simulink library "lib_SecCtrl_Matrices1"  (R2026a)
settings: Solver=VariableStepAuto
undefined symbols (not defined in the file): A_f_sc, A_P_sc, A_Q_sc, A_v_sc, buses_lf, costs2, passM, sec_control_structure
libraries: simulink x3, sl_discontinuities x2
settings Model: Creator=atomas  LastModifiedBy=atomas

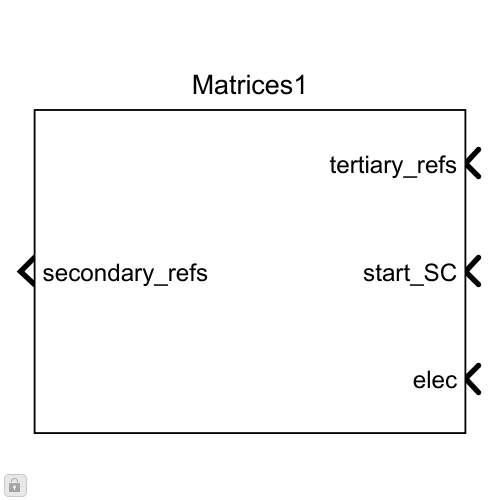
[thumbnail: Simulink's stored preview of the top-level diagram]
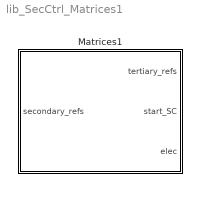
== system lib_SecCtrl_Matrices1 ==
  Matrices1 : Subsystem  VariantControl=Matrices1

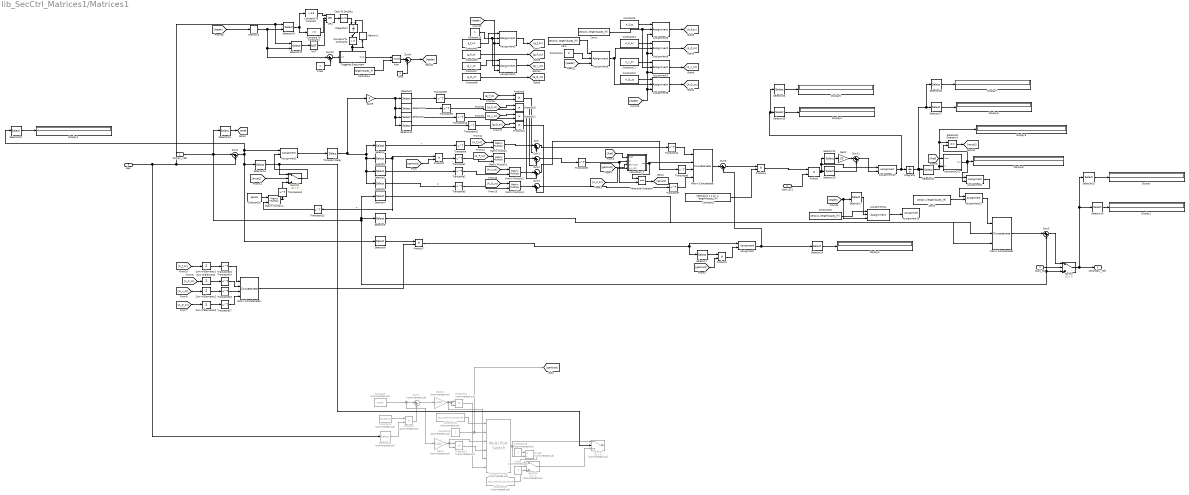
== system lib_SecCtrl_Matrices1/Matrices1 ==
  tertiary_refs : Inport
  start_SC : Inport  Port=2
  elec : Inport  Port=3
  Assignment{,1..2,13} (4 alike) : Assignment  NumberOfDimensions=2  DiagnosticForDimensions=Warning  IndexOptions=Index vector (dialog),Assign all  Indices=2,1  OutputSizes=1,1
  Assignment10 : Assignment  NumberOfDimensions=2  DiagnosticForDimensions=Warning  IndexOptions=Index vector (dialog),Assign all  Indices=1,1  OutputSizes=1,1
  Assignment{3..4,9,11} (4 alike) : Assignment  DiagnosticForDimensions=Warning  IndexOptions=Index vector (port)  Indices=1  OutputSizes=1
  Assignment12 : Assignment  NumberOfDimensions=2  DiagnosticForDimensions=Warning  IndexOptions=Index vector (dialog),Assign all  Indices=1,1  OutputSizes=1,1
  Assignment{5..8} (4 alike) : Assignment  NumberOfDimensions=2  DiagnosticForDimensions=Warning  IndexOptions=Index vector (port),Assign all  Indices=1,1  OutputSizes=1,1
  Cast To Double1 : DataTypeConversion  OutDataTypeStr=double  SaturateOnIntegerOverflow=off  RndMeth=Floor
  Compare To Constant : simulink/Logic and Bit Operations/Compare To Constant  relop=>  const=0.8  OutDataTypeStr=boolean
  Compare To Constant1 : simulink/Logic and Bit Operations/Compare To Constant  relop=<  const=0  OutDataTypeStr=boolean
  Compare To Constant2 : simulink/Logic and Bit Operations/Compare To Constant  relop=>  const=3  OutDataTypeStr=boolean
  Constant : Constant  Commented=on  Value=costs'  VectorParams1D=off
  Constant1 : Constant  Commented=on  Value=2*costs2'  VectorParams1D=off
  Constant10 : Constant  Value=A_P_sc  VectorParams1D=off
  Constant11 : Constant  Value=A_v_sc  VectorParams1D=off
  Constant12 : Constant  Value=A_Q_sc  VectorParams1D=off
  Constant13 : Constant
  Constant14 : Constant  Value=0
  Constant15 : Constant  Value=zeros(1, length(buses_lf))  VectorParams1D=off
  Constant16 : Constant  Commented=on  Value=sec_control_structure
  Constant18 : Constant  Commented=on  Value=sec_control_structure
  Constant19 : Constant  Commented=on  VectorParams1D=off
  Constant2 : Constant  Value=repmat([1 1 1 1]', 1, length(buses_lf))
  Constant20 : Constant  Value=passM  VectorParams1D=off
  Constant3 : Constant  Commented=on
  Constant4 : Constant  Value=length(buses_lf)
  Constant5 : Constant  Value=g_f_sc'  VectorParams1D=off
  Constant6 : Constant  Value=g_P_sc'  VectorParams1D=off
  Constant7 : Constant  Value=g_v_sc'  VectorParams1D=off
  Constant8 : Constant  Value=g_Q_sc'  VectorParams1D=off
  Constant9 : Constant  Value=A_f_sc  VectorParams1D=off
  Display{,1..9} (10 alike) : Display
  Divide : Product  Commented=on  Inputs=*/
  Gain1 : Gain  Commented=on  Gain=1/400
  Gain11 : Gain  Commented=on  Gain=1/400
  Gain2 : Gain  Gain=20
  Gain9 : Gain  Gain=-1
  Integrator : Integrator
  Integrator1 : Integrator  ExternalReset=rising
  Matrix Concatenate : Concatenate  NumInputs=4  Mode=Multidimensional array
  Matrix Concatenate1 : Concatenate  NumInputs=3  Mode=Multidimensional array
  Matrix Concatenate2 : Concatenate  NumInputs=4  Mode=Multidimensional array
  Matrix Multiply{,1..4} (5 alike) : Product  Multiplication=Matrix(*)
  Memory1 : Memory
  Memory2 : Memory  InitialCondition=1
  Mod : Math  Operator=mod
  Multiport Switch : MultiPortSwitch  Commented=on  Inputs=5  SaturateOnIntegerOverflow=off  InputSameDT=off
  NOT : Logic  Operator=NOT  IconShape=distinctive  AllPortsSameDT=off  OutDataTypeStr=boolean
  OR1 : Logic  Operator=OR  Inputs=3  IconShape=distinctive  AllPortsSameDT=off  OutDataTypeStr=boolean
  One : Constant  OutDataTypeStr=Inherit: Inherit via back propagation
  One1 : Constant  OutDataTypeStr=Inherit: Inherit via back propagation
  One3 : Constant  Commented=on  OutDataTypeStr=Inherit: Inherit via back propagation
  Product{,2..4,7,9..12} (9 alike) : Product
  Product1 : Product  Commented=on
  Product13 : Product  Commented=on
  Product14 : Product  Commented=on
  Relational Operator : RelationalOperator  Operator===  OutDataTypeStr=boolean  RndMeth=Simplest  InputSameDT=off
  Relational Operator1 : RelationalOperator  Operator===  OutDataTypeStr=boolean  RndMeth=Simplest  InputSameDT=off
  Selector{,9,19,22,26,28} (6 alike) : Selector  NumberOfDimensions=2  InputPortWidth=3  IndexOptions=Index vector (dialog),Select all  Indices=1,1  OutputSizes=1,1
  Selector{1,7,10,13..15,20..21,23..25,27} (12 alike) : Selector  NumberOfDimensions=2  InputPortWidth=3  IndexOptions=Index vector (dialog),Select all  Indices=2,1  OutputSizes=1,1
  Selector11 : Selector  NumberOfDimensions=2  InputPortWidth=3  IndexOptions=Index vector (dialog),Select all  Indices=4,1  OutputSizes=1,1
  Selector12 : Selector  NumberOfDimensions=2  InputPortWidth=length(buses_lf)  IndexOptions=Index vector (dialog),Index vector (port)  Indices=6,1  OutputSizes=1,1
  Selector16 : Selector  NumberOfDimensions=2  InputPortWidth=length(buses_lf)  IndexOptions=Index vector (dialog),Index vector (port)  Indices=2,1  OutputSizes=1,1
  Selector17 : Selector  NumberOfDimensions=2  InputPortWidth=3  IndexOptions=Index vector (dialog),Index vector (port)  Indices=1,1  OutputSizes=1,1
  Selector18 : Selector  Commented=on  NumberOfDimensions=2  InputPortWidth=3  IndexOptions=Index vector (dialog),Select all  Indices=2,1  OutputSizes=1,1
  Selector2 : Selector  NumberOfDimensions=2  InputPortWidth=3  IndexOptions=Index vector (dialog),Select all  Indices=3,1  OutputSizes=1,1
  Selector3 : Selector  NumberOfDimensions=2  InputPortWidth=3  IndexOptions=Index vector (dialog),Select all  Indices=4,1  OutputSizes=1,1
  Selector4 : Selector  NumberOfDimensions=2  InputPortWidth=3  IndexOptions=Index vector (dialog),Select all  Indices=5,1  OutputSizes=1,1
  Selector5 : Selector  NumberOfDimensions=2  InputPortWidth=3  IndexOptions=Index vector (dialog),Select all  Indices=6,1  OutputSizes=1,1
  Selector6 : Selector  NumberOfDimensions=2  InputPortWidth=3  IndexOptions=Index vector (dialog),Select all  Indices=1:4,1  OutputSizes=1,1
  Selector8 : Selector  NumberOfDimensions=2  InputPortWidth=3  IndexOptions=Index vector (dialog),Select all  Indices=3,1  OutputSizes=1,1
  Sum{,1..3,5,9,11} (7 alike) : Sum  Inputs=|++
  Sum of Elements{,1..3} (4 alike) : Sum  Inputs=+  CollapseMode=Specified dimension  CollapseDim=2
  Sum10 : Sum  Inputs=|+-
  Sum4 : Sum  Inputs=|-+
  Sum6 : Sum  Inputs=|+-
  Sum7 : Sum  Commented=on  Inputs=|++
  Switch : Switch  Criteria=u2 > Threshold  SaturateOnIntegerOverflow=off  InputSameDT=off
  Switch1 : Switch  Criteria=u2 > Threshold  SaturateOnIntegerOverflow=off  InputSameDT=off
  Switch2 : Switch  Commented=on  Criteria=u2 > Threshold  SaturateOnIntegerOverflow=off  InputSameDT=off
  Switch3 : Switch  Commented=on  Criteria=u2 > Threshold  Threshold=1  SaturateOnIntegerOverflow=off  InputSameDT=off
  Transport Delay : TransportDelay  DelayTime=0.1  PadeOrder=3
  Transpose{,1..17} (18 alike) : Math  Operator=transpose
  Triggered Subsystem : Subsystem  TreatAsAtomicUnit=on
  Zero : Constant  Value=zeros(1, length(buses_lf))  VectorParams1D=off  OutDataTypeStr=Inherit: Inherit via back propagation
  Zero1 : Constant  Value=zeros(1, length(buses_lf))  VectorParams1D=off  OutDataTypeStr=Inherit: Inherit via back propagation
  Zero2 : Constant  Value=zeros(1, length(buses_lf))  VectorParams1D=off  OutDataTypeStr=Inherit: Inherit via back propagation
  saturation_P : Subsystem
  saturation_P2 : Subsystem
  start_SC1 : InportShadow  Port=2
  secondary_refs : Outport
  wires:
  Assignment8/1 -> [A_Q_sc]
  Assignment7/1 -> [A_v_sc]
  Assignment6/1 -> [A_P_sc]
  Assignment5/1 -> [A_f_sc]
  Selector27/1 -> Display6/1
  Integrator/1 -> Selector21/1, Assignment1/1, Selector28/1, Selector27/1
  Selector28/1 -> Display7/1
  Selector26/1 -> Display5/1
  Assignment13/1 -> Integrator/1, Selector25/1, Selector26/1
  Selector25/1 -> Display4/1
  [A_P_sc] -> saturation_P/4(A_P_SC)
  Product4/1 -> Product/1
  Selector24/1 -> Display3/1
  Transpose12/1 -> Switch1/3
  Assignment4/1 -> [g_v_sc]
  Assignment3/1 -> [g_f_sc]
  Constant2/1 -> Product4/2
  Assignment1/1 -> Assignment12/1
  [Pref] -> saturation_P2/1(Pref)
  Selector21/1 -> saturation_P2/2(in), Relational Operator1/1, Display9/1
  Relational Operator1/1 -> [awup2]
  saturation_P2/1(out) -> Display8/1, Relational Operator1/2, Assignment1/2
  Sum11/1 -> Assignment13/2
  Sum4/1 -> Selector6/1, Selector14/1, Assignment2/1, Selector20/1
  Selector20/1 -> Display2/1
  Selector23/1 -> Sum11/2
  Product/1 -> Selector23/1, Selector22/1, Assignment13/1
  Gain2/1 -> Sum11/1
  Selector22/1 -> Gain2/1
  Assignment12/1 -> Matrix Concatenate1/1
  Zero2/1 -> Assignment12/2
  Sum1/1 -> Transpose5/1
  Selector19/1 -> Display1/1
  Selector15/1 -> Display/1
  NOT/1 -> OR1/3
  Selector12/1 -> NOT/1
  Assignment2/1 -> Transport Delay/1
  Relational Operator/1 -> [awup1]
  [Pref] -> saturation_P/1(Pref)
  Transpose5/1 -> Relational Operator/2, saturation_P/2(in)
  [gaincost] -> saturation_P/3(gaincost)
  Assignment11/1 -> Assignment10/2
  Sum6/1 -> Product4/1
  Gain9/1 -> Selector9/1, Selector10/1, Selector8/1, Selector11/1
  Sum9/1 -> [leader]
  Switch3/1 -> Switch2/3
  Transpose13/1 -> Matrix Multiply4/2
  [awup1] -> Switch1/2
  Matrix Multiply4/1 -> Transpose12/1
  Constant20/1 -> Matrix Multiply4/1
  tertiary_refs/1 -> Sum5/2, Switch/3, Selector5/1, Selector4/1, Selector13/1, Sum4/1
  Constant19/1 -> Divide/1
  One3/1 -> Switch3/3
  Divide/1 -> Switch3/1
  Constant18/1 -> Switch3/2
  Multiport Switch/1 -> Switch2/1, Divide/2
  Product13/1 -> Multiport Switch/6
  Product14/1 -> Multiport Switch/4
  Gain1/1 -> Product14/1, Product14/2, Multiport Switch/3
  Constant/1 -> Sum7/1, Gain1/1
  Matrix Concatenate1/1 -> Sum5/1
  One1/1 -> Sum10/2
  Sum10/1 -> Triggered Subsystem/1(In1)
  Constant16/1 -> Multiport Switch/1
  Constant3/1 -> Multiport Switch/2, [gaincost]
  Selector18/1 -> Product1/2
  Product1/1 -> Sum7/2
  Gain11/1 -> Product13/1, Product13/2, Multiport Switch/5
  Sum7/1 -> Gain11/1
  Memory1/1 -> Integrator1/2
  OR1/1 -> Cast To Double1/1
  Compare To Constant2/1 -> Triggered Subsystem/Trigger, Memory1/1
  Integrator1/1 -> Compare To Constant2/1
  Constant15/1 -> Assignment11/1
  Selector17/1 -> Assignment11/2
  [leader] -> Selector17/2, Assignment11/3
  Compare To Constant1/1 -> OR1/2
  Compare To Constant/1 -> OR1/1
  [leader] -> Memory2/1
  Constant4/1 -> Mod/2
  Triggered Subsystem/1(Out1) -> Mod/1
  One/1 -> Sum9/2
  Mod/1 -> Sum9/1
  Cast To Double1/1 -> Integrator1/1
  Selector16/1 -> Compare To Constant/1, Compare To Constant1/1
  elec/1 -> Sum4/2, Selector16/1, Selector12/1, Selector18/1
  Memory2/1 -> Selector16/2, Sum10/1, Selector12/2
  Zero1/1 -> Assignment5/2, Assignment7/2
  Assignment9/1 -> Assignment6/2, Assignment8/2
  Zero/1 -> Assignment9/1
  Constant14/1 -> Assignment9/2
  [leader] -> Assignment8/3, Assignment7/3, Assignment6/3, Assignment5/3
  [leader] -> Assignment9/3
  Constant10/1 -> Assignment6/1
  Constant11/1 -> Assignment7/1
  Constant12/1 -> Assignment8/1
  Constant9/1 -> Assignment5/1
  Constant7/1 -> Assignment4/1
  Constant8/1 -> [g_Q_sc]
  Constant6/1 -> [g_P_sc]
  [leader] -> Assignment3/3, Assignment4/3
  Constant13/1 -> Assignment3/2, Assignment4/2
  Constant5/1 -> Assignment3/1
  [g_P_sc] -> Product10/1
  [g_Q_sc] -> Product12/1
  [g_v_sc] -> Product11/1
  [g_f_sc] -> Product9/1
  [A_Q_sc] -> Matrix Multiply3/1
  [A_v_sc] -> Matrix Multiply2/1
  [A_P_sc] -> Matrix Multiply1/1
  [A_f_sc] -> Matrix Multiply/1
  [A_v_sc] -> Sum of Elements2/1
  [A_Q_sc] -> Sum of Elements3/1
  [A_P_sc] -> Sum of Elements/1
  [A_f_sc] -> Sum of Elements1/1
  Matrix Concatenate2/1 -> Product7/2
  Selector6/1 -> Product7/1
  Transpose15/1 -> Matrix Concatenate2/1
  Transpose14/1 -> Matrix Concatenate2/2
  Transpose16/1 -> Matrix Concatenate2/3
  Transpose17/1 -> Matrix Concatenate2/4
  Sum of Elements3/1 -> Transpose17/1
  Sum of Elements2/1 -> Transpose16/1
  Sum of Elements1/1 -> Transpose15/1
  Sum of Elements/1 -> Transpose14/1
  Matrix Multiply/1 -> Sum/1
  Matrix Multiply1/1 -> Sum1/1
  Transpose4/1 -> Matrix Concatenate/1
  Switch1/1 -> Assignment2/2
  Selector14/1 -> Switch1/1, Switch2/2
  Selector13/1 -> [Pref]
  Product3/1 -> Assignment/2
  saturation_P/1(out) -> Relational Operator/1, Matrix Concatenate/2
  Assignment/1 -> Selector24/1, Sum6/2
  Selector7/1 -> Product3/1
  [gaincost] -> Product3/2
  Product7/1 -> Selector7/1, Assignment/1
  [gaincost] -> Product2/2
  Product2/1 -> Transpose1/1
  Constant1/1 -> Product1/1
  Transport Delay/1 -> Gain9/1, Selector/1, Selector1/1, Selector3/1, Selector2/1
  start_SC1/1 -> Product/2
  Matrix Concatenate/1 -> Sum6/1
  Transpose11/1 -> Product12/2
  Transpose10/1 -> Product11/2
  Transpose9/1 -> Product10/2
  Transpose8/1 -> Product9/2
  Sum5/1 -> Switch/1
  Selector11/1 -> Transpose11/1
  Selector10/1 -> Transpose9/1
  Selector9/1 -> Transpose8/1
  Selector5/1 -> Matrix Concatenate1/3
  Switch/1 -> Selector15/1, Selector19/1, secondary_refs/1
  start_SC/1 -> Switch/2
  Selector4/1 -> Matrix Concatenate1/2
  Selector8/1 -> Transpose10/1
  Transpose7/1 -> Matrix Concatenate/4
  Transpose6/1 -> Matrix Concatenate/3
  Transpose3/1 -> Matrix Multiply3/2
  Transpose2/1 -> Matrix Multiply2/2
  Transpose1/1 -> Matrix Multiply1/2
  Transpose/1 -> Matrix Multiply/2
  Matrix Multiply3/1 -> Sum3/1
  Sum3/1 -> Transpose7/1
  Sum2/1 -> Transpose6/1
  Product12/1 -> Sum3/2
  Product11/1 -> Sum2/2
  Matrix Multiply2/1 -> Sum2/1
  Product10/1 -> Sum1/2
  Product9/1 -> Sum/2
  Sum/1 -> Transpose4/1
  Selector2/1 -> Transpose2/1  "v"
  Selector1/1 -> Transpose13/1, Product2/1  "P"
  Selector/1 -> Transpose/1  "f"
  Selector3/1 -> Transpose3/1  "Q"

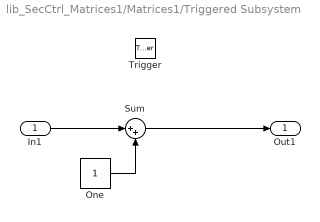
== system lib_SecCtrl_Matrices1/Matrices1/Triggered Subsystem ==
  In1 : Inport
  Trigger : TriggerPort  VariantControl=(inherit)
  One : Constant  OutDataTypeStr=Inherit: Inherit via back propagation
  Sum : Sum  Inputs=|++
  Out1 : Outport
  wires:
  Sum/1 -> Out1/1
  One/1 -> Sum/2
  In1/1 -> Sum/1

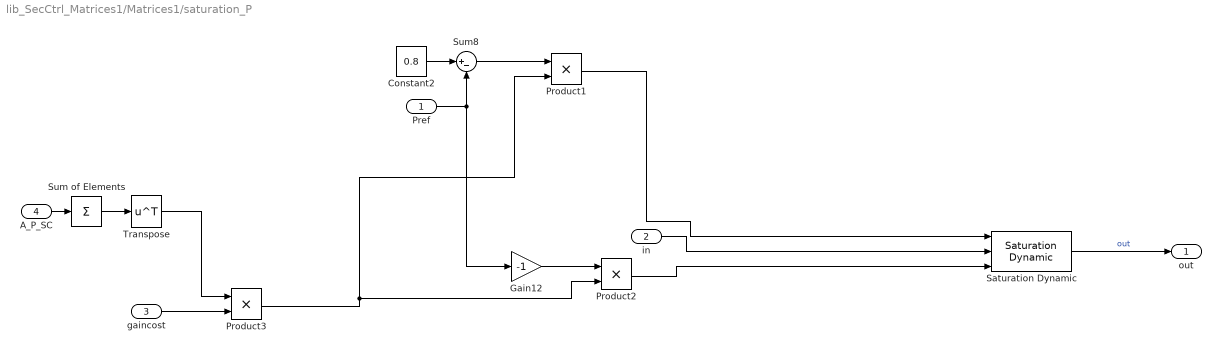
== system lib_SecCtrl_Matrices1/Matrices1/saturation_P ==
  Pref : Inport
  in : Inport  Port=2
  gaincost : Inport  Port=3
  A_P_SC : Inport  Port=4
  Constant2 : Constant  Value=0.8
  Gain12 : Gain  Gain=-1
  Product1 : Product
  Product2 : Product
  Product3 : Product
  Saturation Dynamic : sl_discontinuities/Saturation Dynamic  OutMin=[]  OutMax=[]  OutDataTypeStr=Inherit: Same as second input  OutDataType=fixdt(1, 16)  OutScaling=2^-10  DoSatur=off
  Sum of Elements : Sum  Inputs=+  CollapseMode=Specified dimension  CollapseDim=2
  Sum8 : Sum  Inputs=|+-
  Transpose : Math  Operator=transpose
  out : Outport
  wires:
  Transpose/1 -> Product3/1
  Sum of Elements/1 -> Transpose/1
  gaincost/1 -> Product3/2
  A_P_SC/1 -> Sum of Elements/1
  Gain12/1 -> Product2/1
  Sum8/1 -> Product1/1
  Saturation Dynamic/1 -> out/1  "out"
  Product3/1 -> Product1/2, Product2/2
  in/1 -> Saturation Dynamic/2
  Constant2/1 -> Sum8/1
  Product2/1 -> Saturation Dynamic/3
  Product1/1 -> Saturation Dynamic/1
  Pref/1 -> Gain12/1, Sum8/2

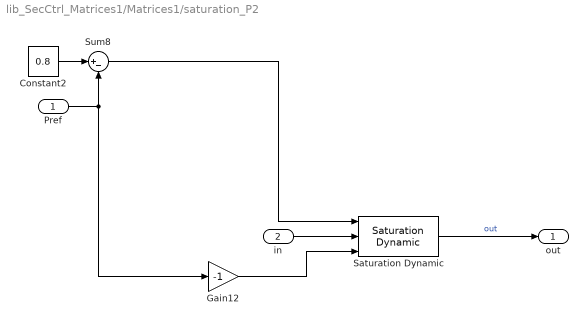
== system lib_SecCtrl_Matrices1/Matrices1/saturation_P2 ==
  Pref : Inport
  in : Inport  Port=2
  Constant2 : Constant  Value=0.8
  Gain12 : Gain  Gain=-1
  Saturation Dynamic : sl_discontinuities/Saturation Dynamic  OutMin=[]  OutMax=[]  OutDataTypeStr=Inherit: Same as second input  OutDataType=fixdt(1, 16)  OutScaling=2^-10  DoSatur=off
  Sum8 : Sum  Inputs=|+-
  out : Outport
  wires:
  Saturation Dynamic/1 -> out/1  "out"
  in/1 -> Saturation Dynamic/2
  Constant2/1 -> Sum8/1
  Gain12/1 -> Saturation Dynamic/3
  Sum8/1 -> Saturation Dynamic/1
  Pref/1 -> Gain12/1, Sum8/2
